simulink model "ECG_GUDB_RPeak_Detector_Frozen"  (R2024b)
settings: Solver=FixedStepDiscrete  StartTime=0.0  StopTime=119.996  FixedStep=0.0040000000000000001  RelTol=1e-3
undefined symbols (not defined in the file): aBP, aHP, aLP, bBP, bHP, bLP, dspblkCoreblockFVToolHelper, Fs, gcbh, Ts
settings Model: Creator=sobha  LastModifiedBy=sobha

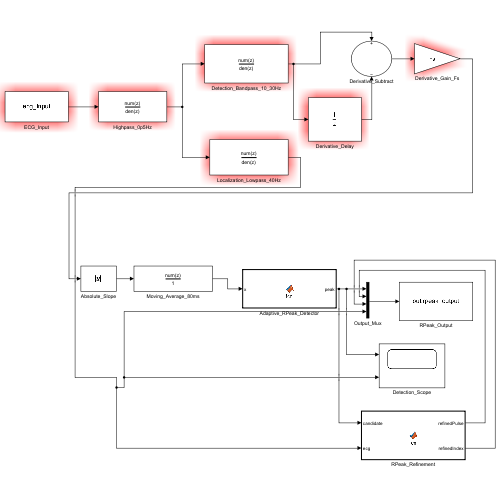
[thumbnail: Simulink's stored preview of the top-level diagram]
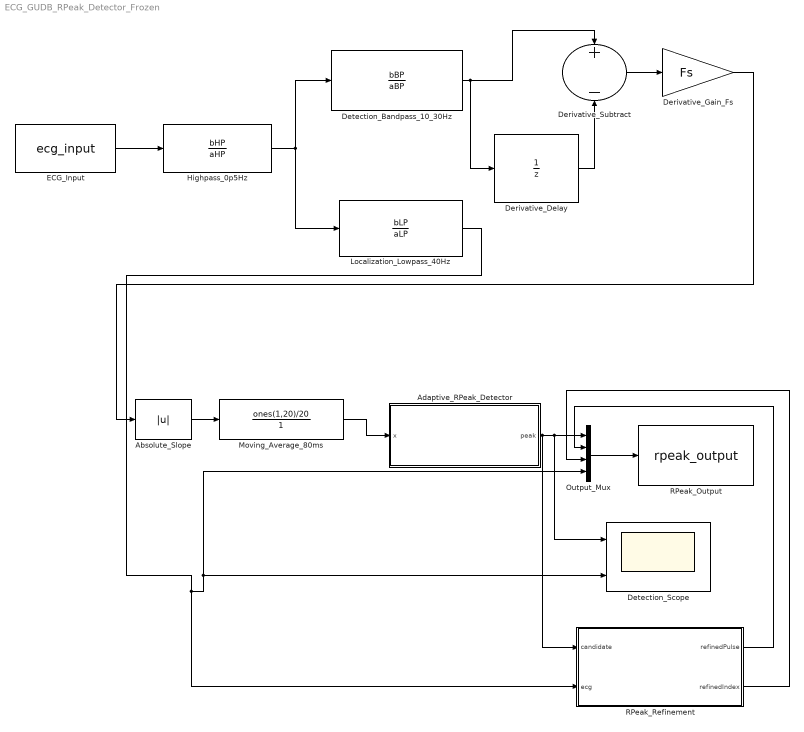
== system ECG_GUDB_RPeak_Detector_Frozen ==
  Absolute_Slope : Abs  SaturateOnIntegerOverflow=off
  Adaptive_RPeak_Detector : MATLAB Function  TreatAsAtomicUnit=on
  Derivative_Delay : UnitDelay  SampleTime=Ts  HasFrameUpgradeWarning=on
  Derivative_Gain_Fs : Gain  Gain=Fs
  Derivative_Subtract : Sum  Inputs=+-
  Detection_Bandpass_10_30Hz : DiscreteFilter  Numerator=bBP  Denominator=aBP
  Detection_Scope : Scope  NumInputPorts=2
  ECG_Input : FromWorkspace  VariableName=ecg_input  SampleTime=Ts
  Highpass_0p5Hz : DiscreteFilter  Numerator=bHP  Denominator=aHP
  Localization_Lowpass_40Hz : DiscreteFilter  Numerator=bLP  Denominator=aLP
  Moving_Average_80ms : DiscreteFilter  LoadFcn=dspblkCoreblockFVToolHelper(gcbh,'load');  Numerator=ones(1,20)/20  Denominator=1
      settings: CopyFcn=dspblkCoreblockFVToolHelper(gcbh,'copy');  DeleteFcn=dspblkCoreblockFVToolHelper(gcbh,'close');  ModelCloseFcn=dspblkCoreblockFVToolHelper(gcbh,'close');  PreSaveFcn=dspblkCoreblockFVToolHelper(gcbh,'presave');  PostSaveFcn=dspblkCoreblockFVToolHelper(gcbh,'postsave');  CloseFcn=dspblkCoreblockFVToolHelper(gcbh,'close');
  Output_Mux : Mux
  RPeak_Output : ToWorkspace  VariableName=rpeak_output  SaveFormat=Timeseries  SampleTime=-1
  RPeak_Refinement : MATLAB Function  TreatAsAtomicUnit=on
  wires:
  ECG_Input/1 -> Highpass_0p5Hz/1
  Highpass_0p5Hz/1 -> Detection_Bandpass_10_30Hz/1, Localization_Lowpass_40Hz/1
  Detection_Bandpass_10_30Hz/1 -> Derivative_Subtract/1, Derivative_Delay/1
  Derivative_Delay/1 -> Derivative_Subtract/2
  Derivative_Subtract/1 -> Derivative_Gain_Fs/1
  Derivative_Gain_Fs/1 -> Absolute_Slope/1
  Absolute_Slope/1 -> Moving_Average_80ms/1
  Moving_Average_80ms/1 -> Adaptive_RPeak_Detector/1(x)
  Adaptive_RPeak_Detector/1(peak) -> Output_Mux/1, Detection_Scope/1, RPeak_Refinement/1(candidate)
  Localization_Lowpass_40Hz/1 -> RPeak_Refinement/2(ecg), Detection_Scope/2, Output_Mux/4
  Output_Mux/1 -> RPeak_Output/1
  RPeak_Refinement/1(refinedPulse) -> Output_Mux/2
  RPeak_Refinement/2(refinedIndex) -> Output_Mux/3

== matlab function ECG_GUDB_RPeak_Detector_Frozen/Adaptive_RPeak_Detector ==
  data: x input; peak output

function peak = fcn(x)
% Rolling-reference adaptive candidate detector
% Fs = 250 Hz

persistent prev2 prev1
persistent sampleCount lastPeak
persistent refBuffer writeIdx

if isempty(sampleCount)
    prev2 = 0;
    prev1 = 0;
    sampleCount = 0;
    lastPeak = -10000;

    % 6-second reference buffer
    refBuffer = zeros(1500,1);
    writeIdx = 1;
end

sampleCount = sampleCount + 1;
peak = 0;

% Update rolling reference buffer
refBuffer(writeIdx) = x;
writeIdx = writeIdx + 1;

if writeIdx > 1500
    writeIdx = 1;
end

% Adaptive threshold
localReference = max(refBuffer);
threshold = 0.35 * localReference;

% Detect local maximum
isLocalMaximum = (prev1 > prev2) && (prev1 >= x);

if isLocalMaximum

    candidateValue = prev1;
    candidateSample = sampleCount - 1;

    % Candidate separation: 120 ms
    % Refractory period: 200 ms
    if candidateValue > threshold && ...
       (candidateSample-lastPeak) >= 50

        peak = 1;
        lastPeak = candidateSample;

    end
end

% Update previous samples
prev2 = prev1;
prev1 = x;

end

== matlab function ECG_GUDB_RPeak_Detector_Frozen/RPeak_Refinement ==
  data: candidate input; refinedPulse output; ecg input; refinedIndex output
function [refinedPulse, refinedIndex] = fcn(candidate, ecg)
%#codegen
% Refine a candidate in a 31-sample ECG window (+/-60 ms at 250 Hz).
persistent n sigBuf pending pendingSample
if isempty(n)
    n = 0;
    sigBuf = zeros(64,1);
    pending = false;
    pendingSample = 0;
end
n = n + 1;
slot = mod(n-1,64) + 1;
sigBuf(slot) = ecg;
refinedPulse = 0;
refinedIndex = 0;
% Candidate pulse is emitted one sample after the envelope maximum.
if candidate > 0.5 && ~pending
    pendingSample = n - 1;
    if pendingSample >= 16
        pending = true;
    end
end
% Wait for 15 future samples, then inspect +/-15 samples around candidate.
if pending && n >= pendingSample + 15
    w = zeros(31,1);
    for k = 1:31
        target = pendingSample - 15 + (k-1);
        readSlot = mod(target-1,64) + 1;
        w(k) = sigBuf(readSlot);
    end
    baseline = median(w);
    [~,iMax] = max(w - baseline);
    [~,iMin] = min(w - baseline);
    if abs(w(iMax)-baseline) >= abs(w(iMin)-baseline)
        refinedOffset = iMax;
    else
        refinedOffset = iMin;
    end
    refinedIndex = pendingSample - 15 + refinedOffset - 1;
    refinedPulse = 1;
    pending = false;
end
end
